simulink model "RoadsterLaunch"  (R2025b)
settings: Solver=ode1  StartTime=0.0  StopTime=8  FixedStep=1e-3  RelTol=1e-3
undefined symbols (not defined in the file): launchMode, rtl
libraries: simulink x1
Description:
  | 0-60 mph. launchMode 0 tyres only, 1 + suction fans, 2 + fans + 2 rear thrusters. Logged: v, x, F_rear, m_air.
settings Model: Creator=kichuiyer  LastModifiedBy=kichuiyer
settings DataIOCC: SaveOutput=off

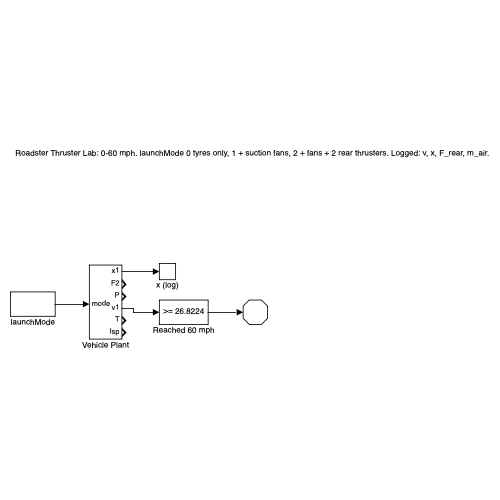
[thumbnail: Simulink's stored preview of the top-level diagram]
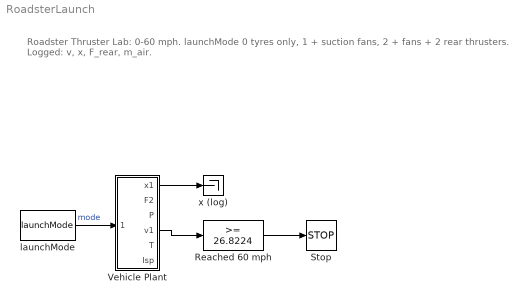
== system RoadsterLaunch ==
  note: Roadster Thruster Lab: 0-60 mph. launchMode 0 tyres only, 1 + suction fans, 2 + fans + 2 rear thrusters. Logged: v, x, F_rear, m_air.
  Reached 60 mph : simulink/Logic and Bit Operations/Compare To Constant  relop=>=  const=26.8224  OutDataTypeStr=boolean
  Stop : Stop
  Vehicle Plant : Subsystem
  launchMode : Constant  Value=launchMode
  x (log) : Terminator
  wires:
  Reached 60 mph/1 -> Stop/1
  Vehicle Plant/1(x1) -> x (log)/1
  Vehicle Plant/4(v1) -> Reached 60 mph/1
  launchMode/1 -> Vehicle Plant/1(mode)  "mode"

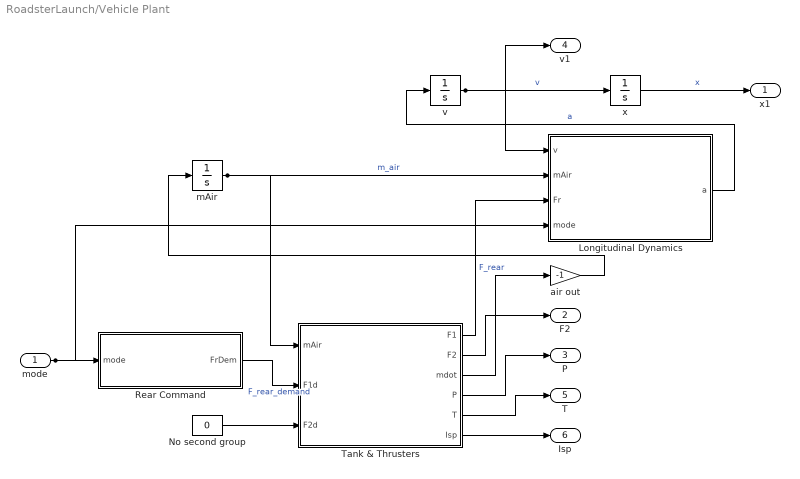
== system RoadsterLaunch/Vehicle Plant ==
  mode : Inport
  Longitudinal Dynamics : MATLAB Function  TreatAsAtomicUnit=on
  No second group : Constant  Value=0
  Rear Command : MATLAB Function  TreatAsAtomicUnit=on
  Tank & Thrusters : MATLAB Function  TreatAsAtomicUnit=on
  air out : Gain  Gain=-1
  mAir : Integrator  InitialCondition=rtl.m0  LimitOutput=on  LowerSaturationLimit=0
  v : Integrator
  x : Integrator
  x1 : Outport
  F2 : Outport  Port=2
  P : Outport  Port=3
  v1 : Outport  Port=4
  T : Outport  Port=5
  Isp : Outport  Port=6
  wires:
  air out/1 -> mAir/1
  Longitudinal Dynamics/1(a) -> v/1  "a"
  x/1 -> x1/1  "x"
  Tank & Thrusters/6(Isp) -> Isp/1
  Tank & Thrusters/4(P) -> P/1
  Tank & Thrusters/5(T) -> T/1
  Tank & Thrusters/2(F2) -> F2/1
  mAir/1 -> Tank & Thrusters/1(mAir), Longitudinal Dynamics/2(mAir)  "m_air"
  Tank & Thrusters/1(F1) -> Longitudinal Dynamics/3(Fr)  "F_rear"
  Rear Command/1(FrDem) -> Tank & Thrusters/2(F1d)  "F_rear_demand"
  v/1 -> v1/1, x/1, Longitudinal Dynamics/1(v)  "v"
  No second group/1 -> Tank & Thrusters/3(F2d)
  Tank & Thrusters/3(mdot) -> air out/1
  mode/1 -> Rear Command/1(mode), Longitudinal Dynamics/4(mode)

== matlab function RoadsterLaunch/Vehicle Plant/Tank & Thrusters ==
  data: mAir input; F1 output; F1d input; F2d input; F2 output; mdot output; P output; T output; Isp output; rtl parameter
function [F1, F2, mdot, P, T, Isp] = tank_thrusters(mAir, F1d, F2d, rtl)
%#codegen
% Cold-gas tank with adiabatic blowdown feeding regulated, choked nozzles.
r   = max(mAir, 1e-6) / rtl.m0;
P   = rtl.P0 * r^rtl.gam;              % isentropic: gas left behind expands
T   = rtl.T0 * r^(rtl.gam - 1);        % ...and cools
pc  = min(rtl.Preg, P);                % regulator caps the nozzle feed
Cf  = rtl.CFm + (pc*rtl.PR - rtl.Pa)/pc*rtl.eps;
Isp = Cf * sqrt(rtl.R*T/rtl.gam) / rtl.CK / rtl.g0;
k   = pc / rtl.Preg;
if pc < 15e5, k = 0; end               % too little pressure to run
F1  = max(F1d, 0) * k;
F2  = max(F2d, 0) * k;
mdot = (F1 + F2) / (Isp * rtl.g0);     % rocket equation: mdot = F/(Isp g0)

== matlab function RoadsterLaunch/Vehicle Plant/Rear Command ==
  data: mode input; FrDem output; rtl parameter
function FrDem = rear_command(mode, rtl)
%#codegen
FrDem = 0;
if mode == 2, FrDem = rtl.FrearMax; end

== matlab function RoadsterLaunch/Vehicle Plant/Longitudinal Dynamics ==
  data: v input; a output; mAir input; Fr input; mode input; rtl parameter
function a = longitudinal(v, mAir, Fr, mode, rtl)
%#codegen
% Tyre force is capped by grip (weight plus fan suction) and by motor power.
m  = rtl.dry + mAir;
dp = 0;
if mode >= 1, dp = rtl.fanKPa*1e3; end
N  = m*rtl.g0 + dp*rtl.fanA;
Ft = min(rtl.mu*N, rtl.motorKW*1e3/max(v, 0.3));
a  = (Ft + Fr - 0.5*1.2*rtl.CdA*v^2 - rtl.crr*N)/m;
